simulink model "interactions"  (R2024b)
settings: Solver=ode23t  StartTime=0.0  StopTime=t_sim  FixedStep=T_sim  MaxStep=1e-4  RelTol=1e-5
values from neighbouring files (symbols this model uses):
  f_b = 50    [init_and_run_perturbed_case.m]    (also in init_emt2.m)
  i_dref1 = 0.0    (= 0)    [init_emt2.m]
  i_dref2 = 0.0    (= 0)    [init_emt2.m]
  i_qref0 = 2.0    (= 2)    [init_emt2.m]
  l_2 = 4e-3    (= 0.004)    [init_emt2.m]
  l_f = 2e-3    (= 0.002)    [init_emt2.m]
  l_g = 3.5e-3    (= 0.0035)    [init_emt2.m]
  params = [w_b, L_f1, L_f2, tau_pll, K_pll, tau_i, K_i]    [init_and_run_perturbed_case.m]    (also in init_emt2.m = [w_b, l_f, kp_i, ki_i, kp_pll_f, ki_pll_f, kp_pll, ki_pll])
  r_2 = 0.2    [init_emt2.m]
  r_f = 0.05    [init_emt2.m]
  r_g = 0.3    [init_emt2.m]
  T_sim = 1e-6    (= 1e-06)    [init_and_run_perturbed_case.m]    (also in init_emt2.m)
  v_b = 380    [init_and_run_perturbed_case.m]    (also in init_emt2.m = 400)
  v_dc = 800    [init_and_run_perturbed_case.m]    (also in init_emt2.m = 700)
libraries: spsThreePhaseSeriesRLCBranchLib x3, spsDCVoltageSourceLib x2, spsThreePhaseVIMeasurementLib x2, spsThreePhaseBreakerLib x2, spsUniversalBridgeLib x2, spsThreePhaseSourceLib x1, sps_lib x1
settings Model: Creator=carlo  LastModifiedBy=carlo
settings DataIOCC: ReturnWorkspaceOutputs=off

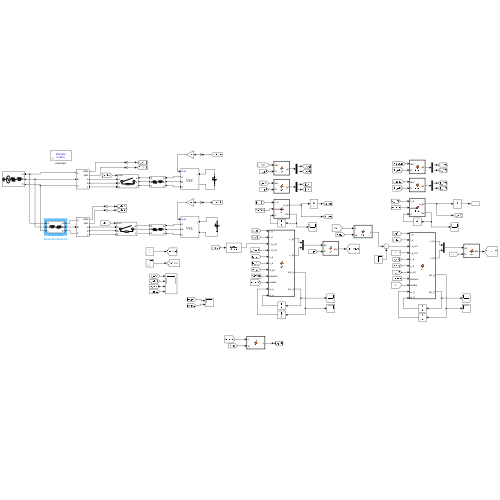
[thumbnail: Simulink's stored preview of the top-level diagram]
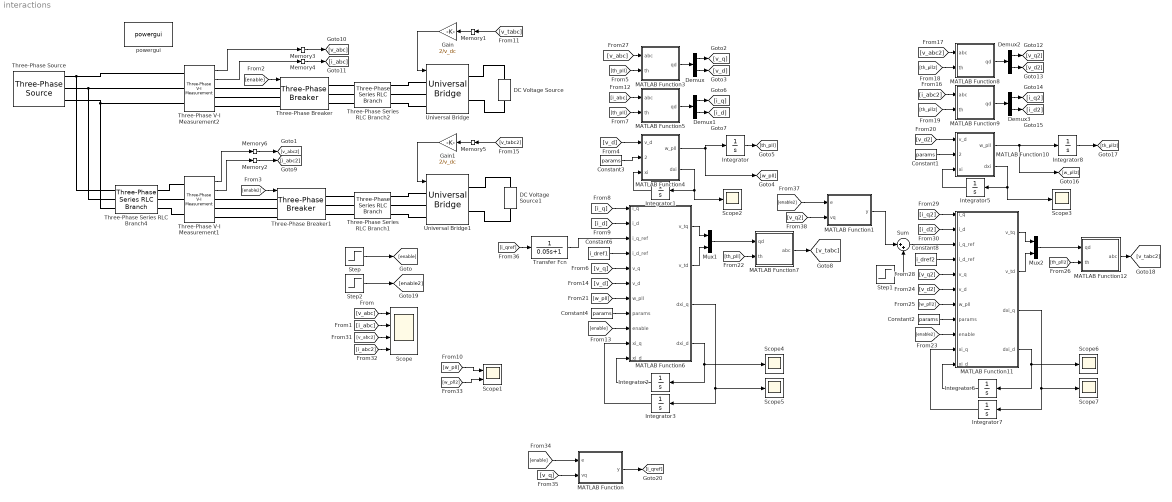
== system interactions ==
  Constant{1..4} (4 alike) : Constant  Value=params
  Constant6 : Constant  Value=i_dref1
  Constant8 : Constant  Value=i_dref2
  DC Voltage Source : spsDCVoltageSourceLib/DC Voltage Source  Amplitude=v_dc  Measurements=None
  DC Voltage Source1 : spsDCVoltageSourceLib/DC Voltage Source  Amplitude=v_dc  Measurements=None
  Demux{,1..3} (4 alike) : Demux  Outputs=2
  Gain : Gain  Gain=2/v_dc
  Gain1 : Gain  Gain=2/v_dc
  Integrator{,1..3,5..8} (8 alike) : Integrator
  MATLAB Function : MATLAB Function  TreatAsAtomicUnit=on
  MATLAB Function1 : MATLAB Function  TreatAsAtomicUnit=on
  MATLAB Function10 : MATLAB Function  TreatAsAtomicUnit=on
  MATLAB Function11 : MATLAB Function  TreatAsAtomicUnit=on
  MATLAB Function12 : MATLAB Function  TreatAsAtomicUnit=on
  MATLAB Function3 : MATLAB Function  TreatAsAtomicUnit=on
  MATLAB Function4 : MATLAB Function  TreatAsAtomicUnit=on
  MATLAB Function5 : MATLAB Function  TreatAsAtomicUnit=on
  MATLAB Function6 : MATLAB Function  TreatAsAtomicUnit=on
  MATLAB Function7 : MATLAB Function  TreatAsAtomicUnit=on
  MATLAB Function8 : MATLAB Function  TreatAsAtomicUnit=on
  MATLAB Function9 : MATLAB Function  TreatAsAtomicUnit=on
  Memory{1..6} (6 alike) : Memory
  Mux1 : Mux  Inputs=2
  Mux2 : Mux  Inputs=2
  Scope : Scope  NumInputPorts=4
  Scope1 : Scope  NumInputPorts=2
  Scope{2..7} (6 alike) : Scope
  Step : Step  Time=0.2  SampleTime=0
  Step1 : Step  Time=10  After=i_qref0  SampleTime=0
  Step2 : Step  Time=0.1  SampleTime=0
  Sum : Sum  Inputs=|++
  Three-Phase Series RLC Branch1 : spsThreePhaseSeriesRLCBranchLib/Three-Phase Series RLC Branch  LConnTagsString=A|B|C  RConnTagsString=A|B|C  BranchType=RL  Resistance=r_f  Inductance=l_f  Capacitance=1e-6  Measurements=None
  Three-Phase Series RLC Branch2 : spsThreePhaseSeriesRLCBranchLib/Three-Phase Series RLC Branch  LConnTagsString=A|B|C  RConnTagsString=A|B|C  BranchType=RL  Resistance=r_f  Inductance=l_f  Capacitance=1e-6  Measurements=None
  Three-Phase Series RLC Branch4 : spsThreePhaseSeriesRLCBranchLib/Three-Phase Series RLC Branch  LConnTagsString=A|B|C  RConnTagsString=A|B|C  BranchType=RL  Resistance=r_2  Inductance=l_2  Capacitance=1e-6  Measurements=None
  Three-Phase V-I Measurement1 : spsThreePhaseVIMeasurementLib/Three-Phase V-I Measurement  VoltageMeasurement=phase-to-ground  SetLabelV=off  LabelV=Vabc  Vpu=off  VpuLL=off  CurrentMeasurement=yes  SetLabelI=off  LabelI=Iabc  Ipu=off  Pbase=100e6  Vbase=500e3  OutputType=Complex  PhasorSimulation=off  PSBequivalent=0
  Three-Phase V-I Measurement2 : spsThreePhaseVIMeasurementLib/Three-Phase V-I Measurement  VoltageMeasurement=phase-to-ground  SetLabelV=off  LabelV=Vabc  Vpu=off  VpuLL=off  CurrentMeasurement=yes  SetLabelI=off  LabelI=Iabc  Ipu=off  Pbase=100e6  Vbase=500e3  OutputType=Complex  PhasorSimulation=off  PSBequivalent=0
  Three-Phase Breaker : spsThreePhaseBreakerLib/Three-Phase Breaker  InitialState=open  SwitchA=on  SwitchB=on  SwitchC=on  SwitchTimes="[1/60  5/60]"  External=on  BreakerResistance=0.01  SnubberResistance=1e6  SnubberCapacitance=inf  Measurements=None
  Three-Phase Breaker1 : spsThreePhaseBreakerLib/Three-Phase Breaker  InitialState=open  SwitchA=on  SwitchB=on  SwitchC=on  SwitchTimes="[1/60  5/60]"  External=on  BreakerResistance=0.01  SnubberResistance=1e6  SnubberCapacitance=inf  Measurements=None
  Three-Phase Source : spsThreePhaseSourceLib/Three-Phase Source  InternalConnection=Yg  VoltagePhases=off  Voltage=v_b  PhaseAngle=0  Voltage_phases=[25e3 25e3 25e3]/sqrt(3)  PhaseAngles_phases=[0 -120 +120]  Frequency=f_b  NonIdealSource=on  SpecifyImpedance=off  Resistance=r_g  Inductance=l_g  ShortCircuitLevel=100e6  BaseVoltage=v_b  XRratio=7  BusType=swing  Pref=10e3  Qref=0  Prefabc=[10e3, 10e3, 10e3]  Qrefabc=[0, 0, 0]  Qmin=-inf  Qmax=inf
  Transfer Fcn : TransferFcn  Denominator=[0.05 1]
  Universal Bridge : spsUniversalBridgeLib/Universal Bridge  Arms=3  SnubberResistance=1e5  SnubberCapacitance=inf  Device=Average-model based VSC  Ron=1e-3  Lon=0  ForwardVoltages="[  0  0  ]"  ForwardVoltage=0  GTOparameters=[ 10e-6 , 20e-6 ]  IGBTparameters=[ 1e-6 , 2e-6 ]  Measurements=None  Measurements_2=None  converterType=Rectifier
  Universal Bridge1 : spsUniversalBridgeLib/Universal Bridge  Arms=3  SnubberResistance=1e5  SnubberCapacitance=inf  Device=Average-model based VSC  Ron=1e-3  Lon=0  ForwardVoltages="[  0  0  ]"  ForwardVoltage=0  GTOparameters=[ 10e-6 , 20e-6 ]  IGBTparameters=[ 1e-6 , 2e-6 ]  Measurements=None  Measurements_2=None  converterType=Rectifier
  powergui : sps_lib/powergui  Priority=1  SimulationMode=Discrete  SampleTime=T_sim  frequency=60  Iterations=50  frequencyindice=0  Pbase=100e6  ErrMax=1e-4  UnitsV=kV  UnitsW=MW  buscounter=0  FunctionMessages=off  echomessages=off  EnableUseOfTLC=off  CurrentSourceSwitches=off  DisableSnubberDevices=off  DisableRonSwitches=off  DisableVfSwitches=off  DisplayEquations=off  AutomaticDiscreteSolvers=off  SolverType=Tustin/Backward Euler (TBE)  Interpol=off  ExternalGateDelay=off  methode=off  Ts=100  x0status=steady  SPID=on  SwTol=0  HookPort=off  NonlinearTolerance=1e-4  nMaxIteration=100  ContinueOnMaxIteration=off  RestoreLinks=warning  ResistiveCurrentMeasurement=off  Frange=[0:2:500]  Ylog=off  Xlog=on  ShowGrid=off  save=off  variable=ZData  structure=0  ZoomFFT=off  StartTime=0.0  cycles=1  DisplayStyle=1  fundamental=60  FreqAxis=off  MaxFrequency=1000  frequencyindicesteady=1  RmsSteady=1  display=off
  wires:
  [v_abc] -> Scope/1
  [i_abc] -> Scope/2
  MATLAB Function5/1(qd) -> Demux1/1
  [v_d] -> MATLAB Function6/6(v_d)
  Constant6/1 -> MATLAB Function6/4(i_d_ref)
  Demux1/1 -> [i_q]
  [i_q] -> MATLAB Function6/1(i_q)
  [i_abc] -> MATLAB Function5/1(abc)
  MATLAB Function4/1(w_pll) -> Integrator/1, [w_pll]
  MATLAB Function6/2(v_td) -> Mux1/2
  [th_pll] -> MATLAB Function7/2(th)
  [i_d] -> MATLAB Function6/2(i_d)
  Constant4/1 -> MATLAB Function6/8(params)
  [v_d] -> MATLAB Function4/1(v_d)
  MATLAB Function3/1(qd) -> Demux/1
  [v_abc] -> MATLAB Function3/1(abc)
  MATLAB Function6/1(v_tq) -> Mux1/1
  Integrator1/1 -> MATLAB Function4/3(xi)
  Demux1/2 -> [i_d]
  [th_pll] -> MATLAB Function3/2(th)
  MATLAB Function4/2(dxi) -> Scope2/1, Integrator1/1
  [w_pll] -> MATLAB Function6/7(w_pll)
  MATLAB Function6/3(dxi_q) -> Scope5/1, Integrator3/1
  [v_q] -> MATLAB Function6/5(v_q)
  Integrator2/1 -> MATLAB Function6/11(xi_d)
  Integrator/1 -> [th_pll]
  Mux1/1 -> MATLAB Function7/1(qd)
  MATLAB Function6/4(dxi_d) -> Scope4/1, Integrator2/1
  Integrator3/1 -> MATLAB Function6/10(xi_q)
  [th_pll] -> MATLAB Function5/2(th)
  Constant3/1 -> MATLAB Function4/2(params)
  MATLAB Function7/1(abc) -> [v_tabc]
  [enable] -> MATLAB Function6/9(enable)
  Memory3/1 -> [v_abc]
  Three-Phase V-I Measurement2/1 -> Memory3/1
  Three-Phase V-I Measurement2/2 -> Memory4/1
  Memory4/1 -> [i_abc]
  [v_tabc] -> Memory1/1
  Memory1/1 -> Gain/1
  Gain/1 -> Universal Bridge/1
  Three-Phase V-I Measurement1/1 -> Memory6/1
  Three-Phase V-I Measurement1/2 -> Memory2/1
  Memory5/1 -> Gain1/1
  [v_tabc2] -> Memory5/1
  Memory6/1 -> [v_abc2]
  Gain1/1 -> Universal Bridge1/1
  [i_abc2] -> MATLAB Function9/1(abc)
  Demux3/1 -> [i_q2]
  MATLAB Function8/1(qd) -> Demux2/1
  Demux3/2 -> [i_d2]
  MATLAB Function9/1(qd) -> Demux3/1
  [th_pll2] -> MATLAB Function8/2(th)
  [th_pll2] -> MATLAB Function9/2(th)
  [v_abc2] -> MATLAB Function8/1(abc)
  Integrator5/1 -> MATLAB Function10/3(xi)
  [v_d2] -> MATLAB Function10/1(v_d)
  MATLAB Function10/2(dxi) -> Scope3/1, Integrator5/1
  Constant1/1 -> MATLAB Function10/2(params)
  [enable2] -> MATLAB Function11/9(enable)
  Constant2/1 -> MATLAB Function11/8(params)
  Integrator6/1 -> MATLAB Function11/11(xi_d)
  [w_pll2] -> MATLAB Function11/7(w_pll)
  [i_d2] -> MATLAB Function11/2(i_d)
  [v_q2] -> MATLAB Function11/5(v_q)
  MATLAB Function11/1(v_tq) -> Mux2/1
  Integrator7/1 -> MATLAB Function11/10(xi_q)
  Mux2/1 -> MATLAB Function12/1(qd)
  [i_q2] -> MATLAB Function11/1(i_q)
  [v_d2] -> MATLAB Function11/6(v_d)
  Constant8/1 -> MATLAB Function11/4(i_d_ref)
  MATLAB Function11/2(v_td) -> Mux2/2
  [th_pll2] -> MATLAB Function12/2(th)
  Step/1 -> [enable]
  MATLAB Function11/4(dxi_d) -> Scope6/1, Integrator6/1
  MATLAB Function11/3(dxi_q) -> Scope7/1, Integrator7/1
  [v_abc2] -> Scope/3
  [i_abc2] -> Scope/4
  Memory2/1 -> [i_abc2]
  [enable] -> Three-Phase Breaker/1
  [enable2] -> Three-Phase Breaker1/1
  MATLAB Function12/1(abc) -> [v_tabc2]
  Sum/1 -> MATLAB Function11/3(i_q_ref)
  Step1/1 -> Sum/2
  [w_pll] -> Scope1/1
  [w_pll2] -> Scope1/2
  Demux/1 -> [v_q]
  Demux/2 -> [v_d]
  Demux2/1 -> [v_q2]
  Demux2/2 -> [v_d2]
  Integrator8/1 -> [th_pll2]
  MATLAB Function10/1(w_pll) -> [w_pll2], Integrator8/1
  Step2/1 -> [enable2]
  MATLAB Function1/1(y) -> Sum/1
  Transfer Fcn/1 -> MATLAB Function6/3(i_q_ref)
  [i_qref] -> Transfer Fcn/1
  [enable] -> MATLAB Function/1(e)
  [v_q] -> MATLAB Function/2(vq)
  MATLAB Function/1(y) -> [i_qref]
  [v_q2] -> MATLAB Function1/2(vq)
  [enable2] -> MATLAB Function1/1(e)
  connections:
  Universal Bridge/LConn2 -- Three-Phase Series RLC Branch2/RConn2
  Three-Phase Series RLC Branch2/RConn1 -- Universal Bridge/LConn1
  Three-Phase Series RLC Branch2/RConn3 -- Universal Bridge/LConn3
  DC Voltage Source/LConn1 -- Universal Bridge/RConn2
  DC Voltage Source/RConn1 -- Universal Bridge/RConn1
  DC Voltage Source1/LConn1 -- Universal Bridge1/RConn2
  DC Voltage Source1/RConn1 -- Universal Bridge1/RConn1
  Three-Phase Series RLC Branch4/RConn3 -- Three-Phase V-I Measurement2/LConn3 -- Three-Phase Source/RConn3
  Three-Phase Series RLC Branch4/LConn2 -- Three-Phase V-I Measurement1/LConn2
  Three-Phase Series RLC Branch4/LConn3 -- Three-Phase V-I Measurement1/LConn3
  Three-Phase Series RLC Branch4/LConn1 -- Three-Phase V-I Measurement1/LConn1
  Three-Phase Series RLC Branch4/RConn1 -- Three-Phase V-I Measurement2/LConn1 -- Three-Phase Source/RConn1
  Three-Phase V-I Measurement2/LConn2 -- Three-Phase Source/RConn2 -- Three-Phase Series RLC Branch4/RConn2
  Three-Phase Series RLC Branch1/RConn3 -- Universal Bridge1/LConn3
  Three-Phase Breaker1/LConn1 -- Three-Phase V-I Measurement1/RConn1
  Three-Phase V-I Measurement1/RConn2 -- Three-Phase Breaker1/LConn2
  Three-Phase Breaker1/LConn3 -- Three-Phase V-I Measurement1/RConn3
  Three-Phase Series RLC Branch1/RConn1 -- Universal Bridge1/LConn1
  Universal Bridge1/LConn2 -- Three-Phase Series RLC Branch1/RConn2
  Three-Phase Breaker/LConn1 -- Three-Phase V-I Measurement2/RConn1
  Three-Phase Breaker/LConn2 -- Three-Phase V-I Measurement2/RConn2
  Three-Phase Breaker/LConn3 -- Three-Phase V-I Measurement2/RConn3
  Three-Phase Breaker/RConn1 -- Three-Phase Series RLC Branch2/LConn1
  Three-Phase Series RLC Branch2/LConn2 -- Three-Phase Breaker/RConn2
  Three-Phase Breaker/RConn3 -- Three-Phase Series RLC Branch2/LConn3
  Three-Phase Breaker1/RConn1 -- Three-Phase Series RLC Branch1/LConn1
  Three-Phase Series RLC Branch1/LConn2 -- Three-Phase Breaker1/RConn2
  Three-Phase Breaker1/RConn3 -- Three-Phase Series RLC Branch1/LConn3

== matlab function interactions/MATLAB Function10 ==
  data: v_d input; w_pll output; params input; xi input; dxi output
function [w_pll, dxi] = fcn(v_d, params, xi)

w_ref = params(1);
kp_pll = params(7);
ki_pll = params(8);

err = v_d;
w_pll = kp_pll*err + xi + w_ref;
dxi = ki_pll*err;

== matlab function interactions/MATLAB Function11 ==
  data: i_q input; i_d input; i_q_ref input; i_d_ref input; v_q input; v_d input; w_pll input; v_tq output; params input; enable input; v_td output; xi_q input; xi_d input; dxi_q output; dxi_d output
function [v_tq, v_td, dxi_q, dxi_d] = fcn(i_q, i_d, i_q_ref, i_d_ref, v_q, v_d, w_pll, params, enable, xi_q, xi_d)

l = params(2);
kp_i = params(3);
ki_i = params(4);

if enable==1
    e_q = i_q_ref - i_q;
    e_d = i_d_ref - i_d;

    u_tq = kp_i*e_q + xi_q;
    u_td = kp_i*e_d + xi_d;

    v_tq = -u_tq - w_pll*l*i_d - v_q;
    v_td = -u_td + w_pll*l*i_q - v_d;

    dxi_q = ki_i*e_q;
    dxi_d = ki_i*e_d;
else
    v_tq = v_q;
    v_td = v_d;
    dxi_q = 0.0;
    dxi_d = 0.0;
end

== matlab function interactions/MATLAB Function12 ==
  data: qd input; abc output; th input
function abc = fcn(qd, th)

Tb = [cos(th),-sin(th);
      cos(th - 2*pi/3),-sin(th - 2*pi/3);
      cos(th + 2*pi/3),-sin(th + 2*pi/3)];
abc = Tb*qd;

== matlab function interactions/MATLAB Function ==
  data: e input; y output; vq input
function y = fcn(e,vq)

y = 2*e*10000/min(max(vq,200),400)/3;

== matlab function interactions/MATLAB Function8 ==
  data: abc input; qd output; th input
function qd = fcn(abc, th)

Tb = 2/3*[cos(th), cos(th - 2*pi/3), cos(th + 2*pi/3);
         -sin(th),-sin(th - 2*pi/3),-sin(th + 2*pi/3)];
qd = Tb*abc;

== matlab function interactions/MATLAB Function1 ==
  data: e input; y output; vq input
function y = fcn(e,vq)

y = 2*e*10000/min(max(vq,200),400)/3;

== matlab function interactions/MATLAB Function3 ==
  data: abc input; qd output; th input
function qd = fcn(abc, th)

Tb = 2/3*[cos(th), cos(th - 2*pi/3), cos(th + 2*pi/3);
         -sin(th),-sin(th - 2*pi/3),-sin(th + 2*pi/3)];
qd = Tb*abc;

== matlab function interactions/MATLAB Function4 ==
  data: v_d input; w_pll output; params input; xi input; dxi output
function [w_pll, dxi] = fcn(v_d, params, xi)

w_ref = params(1);
kp_pll = params(5);
ki_pll = params(6);

err = v_d;
w_pll = kp_pll*err + xi + w_ref;
dxi = ki_pll*err;

== matlab function interactions/MATLAB Function5 ==
  data: abc input; qd output; th input
function qd = fcn(abc, th)

Tb = 2/3*[cos(th), cos(th - 2*pi/3), cos(th + 2*pi/3);
         -sin(th),-sin(th - 2*pi/3),-sin(th + 2*pi/3)];
qd = Tb*abc;

== matlab function interactions/MATLAB Function6 ==
  data: i_q input; i_d input; i_q_ref input; i_d_ref input; v_q input; v_d input; w_pll input; v_tq output; params input; enable input; v_td output; xi_q input; xi_d input; dxi_q output; dxi_d output
function [v_tq, v_td, dxi_q, dxi_d] = fcn(i_q, i_d, i_q_ref, i_d_ref, v_q, v_d, w_pll, params, enable, xi_q, xi_d)

l = params(2);
kp_i = params(3);
ki_i = params(4);

if enable==1
    e_q = i_q_ref - i_q;
    e_d = i_d_ref - i_d;

    u_tq = kp_i*e_q + xi_q;
    u_td = kp_i*e_d + xi_d;

    v_tq = -u_tq - w_pll*l*i_d - v_q;
    v_td = -u_td + w_pll*l*i_q - v_d;

    dxi_q = ki_i*e_q;
    dxi_d = ki_i*e_d;

else
    v_tq = v_q;
    v_td = v_d;
    dxi_q = 0.0;
    dxi_d = 0.0;
end

== matlab function interactions/MATLAB Function7 ==
  data: qd input; abc output; th input
function abc = fcn(qd, th)

Tb = [cos(th),-sin(th);
      cos(th - 2*pi/3),-sin(th - 2*pi/3);
      cos(th + 2*pi/3),-sin(th + 2*pi/3)];
abc = Tb*qd;

== matlab function interactions/MATLAB Function9 ==
  data: abc input; qd output; th input
function qd = fcn(abc, th)

Tb = 2/3*[cos(th), cos(th - 2*pi/3), cos(th + 2*pi/3);
         -sin(th),-sin(th - 2*pi/3),-sin(th + 2*pi/3)];
qd = Tb*abc;
